simulink library "Linkage_Uprights"  (R2025a)
settings: Solver=VariableStepAuto  StartTime=0.0  StopTime=10.0  RelTol=1e-3
undefined symbols (not defined in the file): acamber, atoe, axle_len, axle_mass, axle_whlc_to_bearing, clr_axle, clr_conn_upr, clr_upr, hp_out_c_la, hp_out_f_la, hp_out_f_ua, hp_out_la, hp_out_r_la, hp_out_r_ua, hp_out_ua, hp_pushrod_out, hp_spr_bot, hp_upr_arb, hp_upr_cg, hp_upr_rod, hp_upr_wc, opc_axle, opc_conn_upr, opc_upr, radius_axle, radius_upr, size_conn_upr, upr_mass, whl_init_spd, X, Y, Z
libraries: sm_lib x147, Suspension_Utilities x50, fl_lib x9, nesl_utility x9
(part 1 of 5)
Description:
  | Component of Simscape Vehicle Templates Library
  | 
  | Copyright 2018-2026 The MathWorks, Inc.
settings Model: Creator=smiller  LastModifiedBy=smiller
settings SolverCC: AlgebraicLoopSolver=TrustRegion
settings DataIOCC: ReturnWorkspaceOutputs=off
settings OptimizationCC: ReuseModelBlockBuffer=off
settings DebuggingCC: UnconnectedInputMsg=warning  UnconnectedOutputMsg=warning  UnconnectedLineMsg=warning  ArithmeticOperatorsInVariantConditions=warning
settings ModelReferenceCC: EnableRefExpFcnMdlSchedulingChecks=on
settings SFSimCC: CustomCodeUndefinedFunction=UseInterfaceOnly
settings RTWCC: GPUComputeCapability=3.5

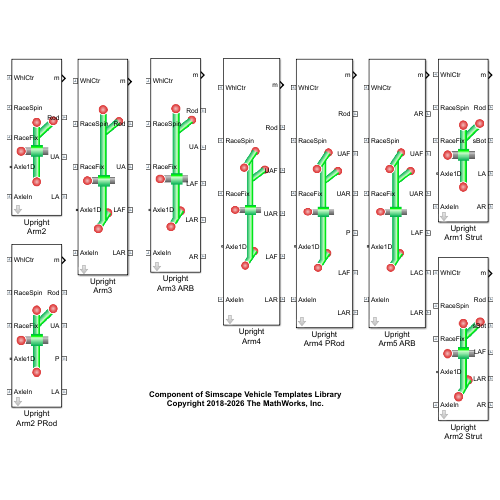
[thumbnail: Simulink's stored preview of the top-level diagram]
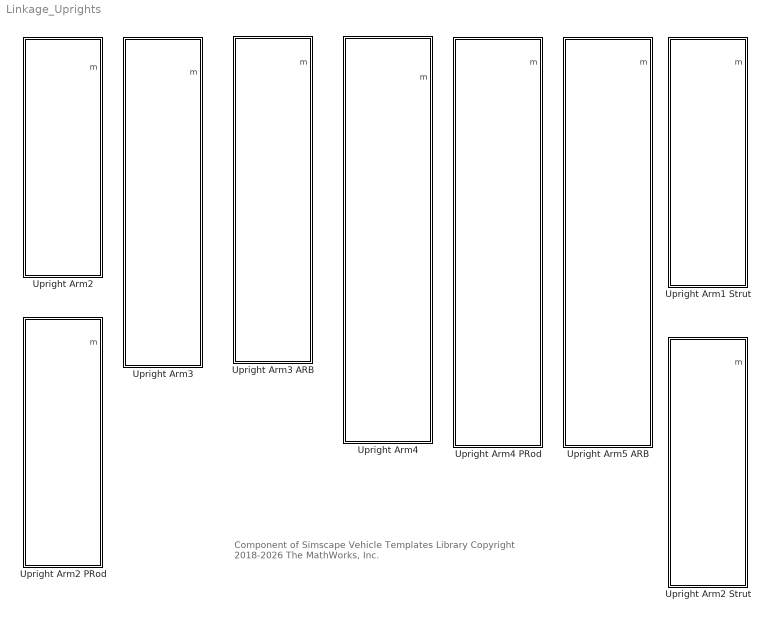
== system Linkage_Uprights ==
  note: Component of Simscape Vehicle Templates Library
      | Copyright 2018-2026 The MathWorks, Inc.
  Upright Arm1 Strut : Subsystem  mask(Upright for One Arm, Steering Rod, and Strut){popup_leftRight=Left, hp_spr_bot=hp_spr_bot, hp_la_out=hp_out_la, hp_upr_rod=hp_upr_rod, hp_upr_arb=hp_upr_arb, hp_upr_cg=hp_upr_cg, hp_upr_wc=hp_upr_wc, axle_len=axle_len, axle_whlc_to_bearing=axle_whlc_to_bearing, axle_mass=axle_mass, atoe=atoe, acamber=acamber, upr_mass=upr_mass, whl_init_spd_upr=whl_init_spd, clr_conn_upr=clr_conn_upr, opc_conn_upr=opc_conn_upr, size_conn_upr=size_conn_upr, clr_upr=clr_upr, opc_upr=opc_upr, radius_upr=radius_upr, clr_axle=clr_axle, opc_axle=opc_axle, radius_axle=radius_axle}
      mask prompts: popup_leftRight "Left/Right"; hp_spr_bot "Spring Bottom [xyz] (m)"; hp_la_out "Lower Arm Outboard [xyz] (m)"; hp_upr_rod "Track Rod Outboard [xyz] (m)"; hp_upr_arb "Anti-Roll Bar [xyz] (m)"; hp_upr_cg "Center of Mass [xyz] (m)"; hp_upr_wc "Wheel Center [xyz] (m)"; axle_len "Axle Length (m)"; axle_whlc_to_bearing "Distance Wheel Ctr to Bearing (m)"; axle_mass "Axle Mass (kg)"; atoe "Toe Angle (deg)"; acamber "Camber Angle (deg)"; upr_mass "Upright Mass (kg)"; whl_init_spd_upr "Initial Wheel Speed (rad/s)"
      mask help: Models an upright (or wheel carrier) that can connect to one arm, steering rod, and a strut. A strut (shock) will typically connect this to the chassis and constrain it to rotate about an axis.
      mask init:
      | % Set parameter for mirroring (+y or -y)
      | if(popup_leftRight == 1)
      |     rhs_upr = 1;
      | elseif(popup_leftRight == 2)
      |     rhs_upr = -1;
      | end
      | rhs_hp = [1 rhs_upr 1];
      | 
      | % Additional hardpoint at center of upright
      | % Used as attachment points for axle and steering arm
      | hp_upr_ctr = (hp_spr_bot+hp_la_out)/2;
      mask TypeOptions popup_leftRight: Left | Right
      mask TypeOptions axle_mass: Axle/Mass
      mask TypeOptions upr_mass:
      | Inertia
      | CG/Mass
      mask TypeOptions whl_init_spd_upr: Revolute/whl_init_spd_jnt
      mask TypeOptions clr_conn_upr:
      | Vis Upright LA/GraphicDiffuseColor | Vis Upright UA/GraphicDiffuseColor | Vis Wheel
      | Center/GraphicDiffuseColor
      mask TypeOptions opc_conn_upr:
      | Vis Upright LA/GraphicOpacity | Vis Upright UA/GraphicOpacity | Vis Wheel
      | Center/GraphicOpacity
      mask TypeOptions clr_upr:
      | Upright/clr_solid | Steering Arm/clr_solid | Bearing
      | Carrier/GraphicDiffuseColor
      mask TypeOptions opc_upr: Upright/opc_solid | Steering Arm/opc_solid
      mask TypeOptions radius_upr: Upright/rad_solid | Steering Arm/rad_solid
      mask TypeOptions clr_axle: Axle/GraphicDiffuseColor
      mask TypeOptions opc_axle: Axle/GraphicOpacity
      mask TypeOptions radius_axle: Axle/CylinderRadius
      mask DialogControl cont_upright Prompt: Upright
      mask DialogControl grp_init Prompt: Initialization
      mask DialogControl cont_vis_upr Prompt: Visualization
      mask DialogControl text_clr_upr Prompt: Color [RGB]
      mask DialogControl text_opc_upr Prompt: Opac. (0-1)
      mask DialogControl text_size_upr Prompt: Size (m)
      mask DialogControl text_conn_upr Prompt: Connections
      mask DialogControl text_upright Prompt: Upright
      mask DialogControl text_stub_axle Prompt: Axle
      mask Display: image('sm_car_vehicle_linkage_dw_upr_IMAGE.png');
  Upright Arm2 : Subsystem  mask(Upright for Two Arms and Steering Rod){popup_leftRight=Left, hp_ua_out=hp_out_ua, hp_la_out=hp_out_la, hp_upr_rod=hp_upr_rod, hp_upr_cg=hp_upr_cg, hp_upr_wc=hp_upr_wc, axle_len=axle_len, axle_whlc_to_bearing=axle_whlc_to_bearing, axle_mass=axle_mass, atoe=atoe, acamber=acamber, upr_mass=upr_mass, whl_init_spd_upr=whl_init_spd, clr_conn_upr=clr_conn_upr, opc_conn_upr=opc_conn_upr, size_conn_upr=size_conn_upr, clr_upr=clr_upr, opc_upr=opc_upr, radius_upr=radius_upr, clr_axle=clr_axle, opc_axle=opc_axle, radius_axle=radius_axle}
      mask prompts: popup_leftRight "Left/Right"; hp_ua_out "Upper Arm Outboard [xyz] (m)"; hp_la_out "Lower Arm Outboard [xyz] (m)"; hp_upr_rod "Track Rod Outboard [xyz] (m)"; hp_upr_cg "Center of Mass [xyz] (m)"; hp_upr_wc "Wheel Center [xyz] (m)"; axle_len "Axle Length (m)"; axle_whlc_to_bearing "Distance Wheel Ctr to Bearing (m)"; axle_mass "Axle Mass (kg)"; atoe "Toe Angle (deg)"; acamber "Camber Angle (deg)"; upr_mass "Upright Mass (kg)"; whl_init_spd_upr "Initial Wheel Speed (rad/s)"
      mask help: Models an upright (or wheel carrier) that can connect to two arms and a steering rod.
      mask init:
      | % Set parameter for mirroring (+y or -y)
      | if(popup_leftRight == 1)
      |     rhs_upr = 1;
      | elseif(popup_leftRight == 2)
      |     rhs_upr = -1;
      | end
      | rhs_hp = [1 rhs_upr 1];
      | 
      | % Additional hardpoint at center of upright
      | % Used as attachment points for axle and steering arm
      | hp_upr_ctr = (hp_ua_out+hp_la_out)/2;
      mask TypeOptions popup_leftRight: Left | Right
      mask TypeOptions axle_mass: Axle/Mass
      mask TypeOptions upr_mass:
      | Inertia
      | CG/Mass
      mask TypeOptions whl_init_spd_upr: Revolute/whl_init_spd_jnt
      mask TypeOptions clr_conn_upr:
      | Vis Upright LA/GraphicDiffuseColor | Vis Upright UA/GraphicDiffuseColor | Vis Wheel
      | Center/GraphicDiffuseColor
      mask TypeOptions opc_conn_upr:
      | Vis Upright LA/GraphicOpacity | Vis Upright UA/GraphicOpacity | Vis Wheel
      | Center/GraphicOpacity
      mask TypeOptions clr_upr: Upright/clr_solid | Steering Arm/clr_solid
      mask TypeOptions opc_upr: Upright/opc_solid | Steering Arm/opc_solid
      mask TypeOptions radius_upr: Upright/rad_solid | Steering Arm/rad_solid
      mask TypeOptions clr_axle: Axle/GraphicDiffuseColor
      mask TypeOptions opc_axle: Axle/GraphicOpacity
      mask TypeOptions radius_axle: Axle/CylinderRadius
      mask DialogControl cont_upright Prompt: Upright
      mask DialogControl grp_upright Prompt: Initialization
      mask DialogControl cont_vis_upr Prompt: Visualization
      mask DialogControl text_clr_upr Prompt: Color [RGB]
      mask DialogControl text_opc_upr Prompt: Opac. (0-1)
      mask DialogControl text_size_upr Prompt: Size (m)
      mask DialogControl text_conn_upr Prompt: Connections
      mask DialogControl text_upright Prompt: Upright
      mask DialogControl text_axle Prompt: Axle
      mask Display: image('sm_car_vehicle_linkage_dw_upr_IMAGE.png');
  Upright Arm2 PRod : Subsystem  mask(Upright for Two Arms, Steering Rod, and Pushrod){popup_leftRight=Left, hp_ua_out=hp_out_ua, hp_la_out=hp_out_la, hp_upr_rod=hp_upr_rod, hp_pushrod=hp_pushrod_out, hp_upr_cg=hp_upr_cg, hp_upr_wc=hp_upr_wc, axle_len=axle_len, axle_whlc_to_bearing=axle_whlc_to_bearing, axle_mass=axle_mass, atoe=atoe, acamber=acamber, upr_mass=upr_mass, whl_init_spd_upr=whl_init_spd, clr_conn_upr=clr_conn_upr, opc_conn_upr=opc_conn_upr, size_conn_upr=size_conn_upr, clr_upr=clr_upr, opc_upr=opc_upr, radius_upr=radius_upr, clr_axle=clr_axle, opc_axle=opc_axle, radius_axle=radius_axle}
      mask prompts: popup_leftRight "Left/Right"; hp_ua_out "Upper Arm Outboard [xyz] (m)"; hp_la_out "Lower Arm Outboard [xyz] (m)"; hp_upr_rod "Track Rod Outboard [xyz] (m)"; hp_pushrod "Pushrod Outboard [xyz] (m)"; hp_upr_cg "Center of Mass [xyz] (m)"; hp_upr_wc "Wheel Center [xyz] (m)"; axle_len "Axle Length (m)"; axle_whlc_to_bearing "Distance Wheel Ctr to Bearing (m)"; axle_mass "Axle Mass (kg)"; atoe "Toe Angle (deg)"; acamber "Camber Angle (deg)"; upr_mass "Upright Mass (kg)"; whl_init_spd_upr "Initial Wheel Speed (rad/s)"
      mask help: Models an upright (or wheel carrier) that can connect to two arms, a steering rod, and a pushrod.
      mask init:
      | % Set parameter for mirroring (+y or -y)
      | if(popup_leftRight == 1)
      |     rhs_upr = 1;
      | elseif(popup_leftRight == 2)
      |     rhs_upr = -1;
      | end
      | rhs_hp = [1 rhs_upr 1];
      | 
      | % Additional hardpoint at center of upright
      | % Used as attachment points for axle and steering arm
      | hp_upr_ctr = (hp_ua_out+hp_la_out)/2;
      mask TypeOptions popup_leftRight: Left | Right
      mask TypeOptions axle_mass: Axle/Mass
      mask TypeOptions upr_mass:
      | Inertia
      | CG/Mass
      mask TypeOptions whl_init_spd_upr: Revolute/whl_init_spd_jnt
      mask TypeOptions clr_conn_upr:
      | Vis Upright LA/GraphicDiffuseColor | Vis Upright UA/GraphicDiffuseColor | Vis Wheel
      | Center/GraphicDiffuseColor
      mask TypeOptions opc_conn_upr:
      | Vis Upright LA/GraphicOpacity | Vis Upright UA/GraphicOpacity | Vis Wheel
      | Center/GraphicOpacity
      mask TypeOptions clr_upr:
      | Upright/clr_solid | Steering Arm/clr_solid | Bearing
      | Carrier/GraphicDiffuseColor | Pushrod Conn/clr_solid
      mask TypeOptions opc_upr: Upright/opc_solid | Steering Arm/opc_solid | Pushrod Conn/opc_solid
      mask TypeOptions radius_upr: Upright/rad_solid | Steering Arm/rad_solid | Pushrod Conn/rad_solid
      mask TypeOptions clr_axle: Axle/GraphicDiffuseColor
      mask TypeOptions opc_axle: Axle/GraphicOpacity
      mask TypeOptions radius_axle: Axle/CylinderRadius
      mask DialogControl cont_upright Prompt: Upright
      mask DialogControl grp_init Prompt: Initialization
      mask DialogControl cont_vis_upr Prompt: Visualization
      mask DialogControl text_clr_upr Prompt: Color [RGB]
      mask DialogControl text_opc_upr Prompt: Opac. (0-1)
      mask DialogControl text_size_upr Prompt: Size (m)
      mask DialogControl text_conn_upr Prompt: Connections
      mask DialogControl text_upright Prompt: Upright
      mask DialogControl text_stub_axle Prompt: Axle
      mask Display: image('sm_car_vehicle_linkage_dw_upr_IMAGE.png');
  Upright Arm2 Strut : Subsystem  mask(Upright for Two Arms, Steering Rod, and Strut){popup_leftRight=Left, hp_spr_bot=hp_spr_bot, hp_laf_out=hp_out_f_la, hp_lar_out=hp_out_r_la, hp_upr_rod=hp_upr_rod, hp_upr_arb=hp_upr_arb, hp_upr_cg=hp_upr_cg, hp_upr_wc=hp_upr_wc, axle_len=axle_len, axle_whlc_to_bearing=axle_whlc_to_bearing, axle_mass=axle_mass, atoe=atoe, acamber=acamber, upr_mass=upr_mass, whl_init_spd_upr=whl_init_spd, clr_conn_upr=clr_conn_upr, opc_conn_upr=opc_conn_upr, size_conn_upr=size_conn_upr, clr_upr=clr_upr, opc_upr=opc_upr, radius_upr=radius_upr, clr_axle=clr_axle, opc_axle=opc_axle, radius_axle=radius_axle}
      mask prompts: popup_leftRight "Left/Right"; hp_spr_bot "Spring Bottom [xyz] (m)"; hp_laf_out "Lower Arm Front Outboard [xyz] (m)"; hp_lar_out "Lower Arm Rear Outboard [xyz] (m)"; hp_upr_rod "Track Rod Outboard [xyz] (m)"; hp_upr_arb "Anti-Roll Bar [xyz] (m)"; hp_upr_cg "Center of Mass [xyz] (m)"; hp_upr_wc "Wheel Center [xyz] (m)"; axle_len "Axle Length (m)"; axle_whlc_to_bearing "Distance Wheel Ctr to Bearing (m)"; axle_mass "Axle Mass (kg)"; atoe "Toe Angle (deg)"; acamber "Camber Angle (deg)"; upr_mass "Upright Mass (kg)"; whl_init_spd_upr "Initial Wheel Speed (rad/s)"
      mask help: Models an upright (or wheel carrier) that can connect to two arms, steering rod, and a strut. A strut (shock) will typically connect this to the chassis and constrain it to rotate about an axis.
      mask init:
      | % Set parameter for mirroring (+y or -y)
      | if(popup_leftRight == 1)
      |     rhs_upr = 1;
      | elseif(popup_leftRight == 2)
      |     rhs_upr = -1;
      | end
      | rhs_hp = [1 rhs_upr 1];
      | 
      | % Additional hardpoint at center of upright
      | % Used as attachment points for axle and steering arm
      | hp_upr_ctr = (hp_spr_bot+hp_laf_out)/2;
      mask TypeOptions popup_leftRight: Left | Right
      mask TypeOptions axle_mass: Axle/Mass
      mask TypeOptions upr_mass:
      | Inertia
      | CG/Mass
      mask TypeOptions whl_init_spd_upr: Revolute/whl_init_spd_jnt
      mask TypeOptions clr_conn_upr:
      | Vis Upright LA/GraphicDiffuseColor | Vis Upright UA/GraphicDiffuseColor | Vis Wheel
      | Center/GraphicDiffuseColor
      mask TypeOptions opc_conn_upr:
      | Vis Upright LA/GraphicOpacity | Vis Upright UA/GraphicOpacity | Vis Wheel
      | Center/GraphicOpacity
      mask TypeOptions clr_upr:
      | Upright/clr_solid | Steering Arm/clr_solid | Bearing
      | Carrier/GraphicDiffuseColor
      mask TypeOptions opc_upr: Upright/opc_solid | Steering Arm/opc_solid
      mask TypeOptions radius_upr: Upright/rad_solid | Steering Arm/rad_solid
      mask TypeOptions clr_axle: Axle/GraphicDiffuseColor
      mask TypeOptions opc_axle: Axle/GraphicOpacity
      mask TypeOptions radius_axle: Axle/CylinderRadius
      mask DialogControl cont_upright Prompt: Upright
      mask DialogControl grp_init Prompt: Initialization
      mask DialogControl cont_vis_upr Prompt: Visualization
      mask DialogControl text_clr_upr Prompt: Color [RGB]
      mask DialogControl text_opc_upr Prompt: Opac. (0-1)
      mask DialogControl text_size_upr Prompt: Size (m)
      mask DialogControl text_conn_upr Prompt: Connections
      mask DialogControl text_upright Prompt: Upright
      mask DialogControl text_stub_axle Prompt: Axle
      mask Display: image('sm_car_vehicle_linkage_sla_arb_IMAGE.png');
  Upright Arm3 : Subsystem  mask(Upright for Three Arms and Steering Rod){popup_leftRight=Left, hp_ua_out=hp_out_ua, hp_laf_out=hp_out_f_la, hp_lar_out=hp_out_r_la, hp_upr_rod=hp_upr_rod, hp_upr_cg=hp_upr_cg, hp_upr_wc=hp_upr_wc, axle_len=axle_len, axle_whlc_to_bearing=axle_whlc_to_bearing, axle_mass=axle_mass, atoe=atoe, acamber=acamber, upr_mass=upr_mass, whl_init_spd_upr=whl_init_spd, clr_conn_upr=clr_conn_upr, opc_conn_upr=opc_conn_upr, size_conn_upr=size_conn_upr, clr_upr=clr_upr, opc_upr=opc_upr, radius_upr=radius_upr, clr_axle=clr_axle, opc_axle=opc_axle, radius_axle=radius_axle}
      mask prompts: popup_leftRight "Left/Right"; hp_ua_out "Upper Arm Outboard [xyz] (m)"; hp_laf_out "Lower Front Arm Outboard [xyz] (m)"; hp_lar_out "Lower Rear Arm Outboard [xyz] (m)"; hp_upr_rod "Track Rod Outboard [xyz] (m)"; hp_upr_cg "Center of Mass [xyz] (m)"; hp_upr_wc "Wheel Center [xyz] (m)"; axle_len "Axle Length(m)"; axle_whlc_to_bearing "Distance Wheel Ctr to Bearing (m)"; axle_mass "Axle Mass (kg)"; atoe "Toe Angle (deg)"; acamber "Camber Angle (deg)"; upr_mass "Upright Mass (kg)"; whl_init_spd_upr "Initial Wheel Speed (rad/s)"
      mask help: Models an upright (or wheel carrier) that can connect to three arms and a steering rod.
      mask init:
      | % Set parameter for mirroring (+y or -y)
      | if(popup_leftRight == 1)
      |     rhs_upr = 1;
      | elseif(popup_leftRight == 2)
      |     rhs_upr = -1;
      | end
      | rhs_hp = [1 rhs_upr 1];
      | 
      | % Additional hardpoint at center of upright
      | % Used as attachment points for axle and steering arm
      | hp_upr_ctr = (hp_ua_out+hp_laf_out)/2;
      mask TypeOptions popup_leftRight: Left | Right
      mask TypeOptions axle_mass: Axle/Mass
      mask TypeOptions upr_mass:
      | Inertia
      | CG/Mass
      mask TypeOptions whl_init_spd_upr: Revolute/whl_init_spd_jnt
      mask TypeOptions clr_conn_upr:
      | Vis Upright LAF/GraphicDiffuseColor | Vis Upright UAF/GraphicDiffuseColor | Vis Wheel
      | Center/GraphicDiffuseColor
      mask TypeOptions opc_conn_upr:
      | Vis Upright LAF/GraphicOpacity | Vis Upright UAF/GraphicOpacity | Vis Wheel
      | Center/GraphicOpacity
      mask TypeOptions clr_upr: Upright/clr_solid | Steering Arm/clr_solid
      mask TypeOptions opc_upr: Upright/opc_solid | Steering Arm/opc_solid
      mask TypeOptions radius_upr: Upright/rad_solid | Steering Arm/rad_solid
      mask TypeOptions clr_axle: Axle/GraphicDiffuseColor
      mask TypeOptions opc_axle: Axle/GraphicOpacity
      mask TypeOptions radius_axle: Axle/CylinderRadius
      mask DialogControl cont_upright Prompt: Upright
      mask DialogControl grp_upright Prompt: Upright
      mask DialogControl cont_vis_upr Prompt: Visualization
      mask DialogControl text_clr_upr Prompt: Color [RGB]
      mask DialogControl text_opc_upr Prompt: Opac. (0-1)
      mask DialogControl text_size_upr Prompt: Size (m)
      mask DialogControl text_conn_upr Prompt: Connections
      mask DialogControl text_upright Prompt: Upright
      mask DialogControl text_axle Prompt: Axle
      mask Display: image('sm_car_vehicle_linkage_sla_upr_IMAGE.png');
  Upright Arm3 ARB : Subsystem  mask(Upright for Three Arms, Steering Rod, Anti-Roll Bar){popup_leftRight=Left, hp_ua_out=hp_out_ua, hp_laf_out=hp_out_f_la, hp_lar_out=hp_out_r_la, hp_upr_rod=hp_upr_rod, hp_upr_arb=hp_upr_arb, hp_upr_cg=hp_upr_cg, hp_upr_wc=hp_upr_wc, axle_len=axle_len, axle_whlc_to_bearing=axle_whlc_to_bearing, axle_mass=axle_mass, atoe=atoe, acamber=acamber, upr_mass=upr_mass, whl_init_spd_upr=whl_init_spd, clr_conn_upr=clr_conn_upr, opc_conn_upr=opc_conn_upr, size_conn_upr=size_conn_upr, clr_upr=clr_upr, opc_upr=opc_upr, radius_upr=radius_upr, clr_axle=clr_axle, opc_axle=opc_axle, radius_axle=radius_axle}
      mask prompts: popup_leftRight "Left/Right"; hp_ua_out "Upper Arm Outboard [xyz] (m)"; hp_laf_out "Lower Front Arm Outboard [xyz] (m)"; hp_lar_out "Lower Rear Arm Outboard [xyz] (m)"; hp_upr_rod "Track Rod Outboard [xyz] (m)"; hp_upr_arb "Anti-Roll Bar [xyz] (m)"; hp_upr_cg "Center of Mass [xyz] (m)"; hp_upr_wc "Wheel Center [xyz] (m)"; axle_len "Axle Length(m)"; axle_whlc_to_bearing "Distance Wheel Ctr to Bearing (m)"; axle_mass "Axle Mass (kg)"; atoe "Toe Angle (deg)"; acamber "Camber Angle (deg)"; upr_mass "Upright Mass (kg)"; whl_init_spd_upr "Initial Wheel Speed (rad/s)"
      mask help: Models an upright (or wheel carrier) that can connect to three arms, a steering rod and an anti-roll bar.
      mask init: same as Linkage_Uprights/Upright Arm3
      mask TypeOptions popup_leftRight: Left | Right
      mask TypeOptions axle_mass: Axle/Mass
      mask TypeOptions upr_mass:
      | Inertia
      | CG/Mass
      mask TypeOptions whl_init_spd_upr: Revolute/whl_init_spd_jnt
      mask TypeOptions clr_conn_upr:
      | Vis Upright LAF/GraphicDiffuseColor | Vis Upright UAF/GraphicDiffuseColor | Vis Wheel
      | Center/GraphicDiffuseColor
      mask TypeOptions opc_conn_upr:
      | Vis Upright LAF/GraphicOpacity | Vis Upright UAF/GraphicOpacity | Vis Wheel
      | Center/GraphicOpacity
      mask TypeOptions clr_upr: Upright/clr_solid | Steering Arm/clr_solid
      mask TypeOptions opc_upr: Upright/opc_solid | Steering Arm/opc_solid
      mask TypeOptions radius_upr: Upright/rad_solid | Steering Arm/rad_solid
      mask TypeOptions clr_axle: Axle/GraphicDiffuseColor
      mask TypeOptions opc_axle: Axle/GraphicOpacity
      mask TypeOptions radius_axle: Axle/CylinderRadius
      mask DialogControl cont_upright Prompt: Upright
      mask DialogControl grp_upright Prompt: Upright
      mask DialogControl cont_vis_upr Prompt: Visualization
      mask DialogControl text_clr_upr Prompt: Color [RGB]
      mask DialogControl text_opc_upr Prompt: Opac. (0-1)
      mask DialogControl text_size_upr Prompt: Size (m)
      mask DialogControl text_conn_upr Prompt: Connections
      mask DialogControl text_upright Prompt: Upright
      mask DialogControl text_axle Prompt: Axle
      mask Display: image('sm_car_vehicle_linkage_sla_upr_IMAGE.png');
  Upright Arm4 : Subsystem  mask(Upright for Four Arms and Steering Rod){popup_leftRight=Left, hp_uaf_out=hp_out_f_ua, hp_uar_out=hp_out_r_ua, hp_laf_out=hp_out_f_la, hp_lar_out=hp_out_r_la, hp_upr_rod=hp_upr_rod, hp_upr_cg=hp_upr_cg, hp_upr_wc=hp_upr_wc, axle_len=axle_len, axle_whlc_to_bearing=axle_whlc_to_bearing, axle_mass=axle_mass, atoe=atoe, acamber=acamber, upr_mass=upr_mass, whl_init_spd_upr=whl_init_spd, clr_conn_upr=clr_conn_upr, opc_conn_upr=opc_conn_upr, size_conn_upr=size_conn_upr, clr_upr=clr_upr, opc_upr=opc_upr, radius_upr=radius_upr, clr_axle=clr_axle, opc_axle=opc_axle, radius_axle=radius_axle}
      mask prompts: popup_leftRight "Left/Right"; hp_uaf_out "Upper Arm Front Outboard [xyz] (m)"; hp_uar_out "Upper Arm Rear Outboard [xyz] (m)"; hp_laf_out "Lower Arm Front Outboard [xyz] (m)"; hp_lar_out "Lower Arm Rear Outboard [xyz] (m)"; hp_upr_rod "Track Rod Outboard [xyz] (m)"; hp_upr_cg "Center of Mass [xyz] (m)"; hp_upr_wc "Wheel Center [xyz] (m)"; axle_len "Axle Length (m)"; axle_whlc_to_bearing "Distance Wheel Ctr to Bearing (m)"; axle_mass "Axle Mass (kg)"; atoe "Toe Angle (deg)"; acamber "Camber Angle (deg)"; upr_mass "Upright Mass (kg)"; whl_init_spd_upr "Initial Wheel Speed (rad/s)"
      mask help: Models an upright (or wheel carrier) that can connect to four arms and a steering rod.
      mask init:
      | % Set parameter for mirroring (+y or -y)
      | if(popup_leftRight == 1)
      |     rhs_upr = 1;
      | elseif(popup_leftRight == 2)
      |     rhs_upr = -1;
      | end
      | rhs_hp = [1 rhs_upr 1];
      | 
      | % Additional hardpoint at center of upright
      | % Used as attachment points for axle and steering arm
      | hp_upr_ctr = (hp_uaf_out+hp_laf_out)/2;
      mask TypeOptions popup_leftRight: Left | Right
      mask TypeOptions axle_mass: Axle/Mass
      mask TypeOptions upr_mass:
      | Inertia
      | CG/Mass
      mask TypeOptions whl_init_spd_upr: Revolute/whl_init_spd_jnt
      mask TypeOptions clr_conn_upr:
      | Vis Upright LAF/GraphicDiffuseColor | Vis Upright UAF/GraphicDiffuseColor | Vis
      | Wheel
      | Center/GraphicDiffuseColor
      mask TypeOptions opc_conn_upr:
      | Vis Upright LAF/GraphicOpacity | Vis Upright UAF/GraphicOpacity | Vis
      | Wheel
      | Center/GraphicOpacity
      mask TypeOptions clr_upr: Upright/clr_solid | Steering Arm/clr_solid
      mask TypeOptions opc_upr: Upright/opc_solid | Steering Arm/opc_solid
      mask TypeOptions radius_upr: Upright/rad_solid | Steering Arm/rad_solid
      mask TypeOptions clr_axle: Axle/GraphicDiffuseColor
      mask TypeOptions opc_axle: Axle/GraphicOpacity
      mask TypeOptions radius_axle: Axle/CylinderRadius
      mask DialogControl cont_upright Prompt: Upright
      mask DialogControl grp_upright Prompt: Initialization
      mask DialogControl cont_vis_upr Prompt: Visualization
      mask DialogControl text_clr_upr Prompt: Color [RGB]
      mask DialogControl text_opc_upr Prompt: Opac. (0-1)
      mask DialogControl text_size_upr Prompt: Size (m)
      mask DialogControl text_conn_upr Prompt: Connections
      mask DialogControl text_upright Prompt: Upright
      mask DialogControl text_axle Prompt: Axle
      mask Display: image('sm_car_vehicle_linkage_link5_upr_IMAGE.png');
  Upright Arm4 PRod : Subsystem  mask(Upright for Four Arms, Steering Rod, and Pushrod){popup_leftRight=Left, hp_uaf_out=hp_out_f_ua, hp_uar_out=hp_out_r_ua, hp_laf_out=hp_out_f_la, hp_lar_out=hp_out_r_la, hp_pushrod=hp_pushrod_out, hp_upr_rod=hp_upr_rod, hp_upr_cg=hp_upr_cg, hp_upr_wc=hp_upr_wc, axle_len=axle_len, axle_whlc_to_bearing=axle_whlc_to_bearing, axle_mass=axle_mass, atoe=atoe, acamber=acamber, upr_mass=upr_mass, whl_init_spd_upr=whl_init_spd, clr_conn_upr=clr_conn_upr, opc_conn_upr=opc_conn_upr, size_conn_upr=size_conn_upr, clr_upr=clr_upr, opc_upr=opc_upr, radius_upr=radius_upr, clr_axle=clr_axle, opc_axle=opc_axle, radius_axle=radius_axle}
      mask prompts: popup_leftRight "Left/Right"; hp_uaf_out "Upper Arm Front Outboard [xyz] (m)"; hp_uar_out "Upper Arm Rear Outboard [xyz] (m)"; hp_laf_out "Lower Arm Front Outboard [xyz] (m)"; hp_lar_out "Lower Arm Rear Outboard [xyz] (m)"; hp_pushrod "Pushrod Outboard [xyz] (m)"; hp_upr_rod "Track Rod Outboard [xyz] (m)"; hp_upr_cg "Center of Mass [xyz] (m)"; hp_upr_wc "Wheel Center [xyz] (m)"; axle_len "Axle Length (m)"; axle_whlc_to_bearing "Distance Wheel Ctr to Bearing (m)"; axle_mass "Axle Mass (kg)"; atoe "Toe Angle (deg)"; acamber "Camber Angle (deg)"; upr_mass "Upright Mass (kg)"; whl_init_spd_upr "Initial Wheel Speed (rad/s)"
      mask help: Models an upright (or wheel carrier) that can connect to four arms, a steering rod, and a pushrod.
      mask init: same as Linkage_Uprights/Upright Arm4
      mask TypeOptions popup_leftRight: Left | Right
      mask TypeOptions axle_mass: Axle/Mass
      mask TypeOptions upr_mass:
      | Inertia
      | CG/Mass
      mask TypeOptions whl_init_spd_upr: Revolute/whl_init_spd_jnt
      mask TypeOptions clr_conn_upr:
      | Vis Upright LAF/GraphicDiffuseColor | Vis Upright UAF/GraphicDiffuseColor | Vis
      | Wheel
      | Center/GraphicDiffuseColor
      mask TypeOptions opc_conn_upr:
      | Vis Upright LAF/GraphicOpacity | Vis Upright UAF/GraphicOpacity | Vis
      | Wheel
      | Center/GraphicOpacity
      mask TypeOptions clr_upr:
      | Upright/clr_solid | Steering Arm/clr_solid | Lower
      | Rear Arm/clr_solid | Upper
      | Rear Arm/clr_solid | Pushrod Conn/clr_solid
      mask TypeOptions opc_upr:
      | Upright/opc_solid | Steering Arm/opc_solid | Lower
      | Rear Arm/opc_solid | Upper
      | Rear Arm/opc_solid | Pushrod Conn/opc_solid
      mask TypeOptions radius_upr:
      | Upright/rad_solid | Steering Arm/rad_solid | Lower
      | Rear Arm/rad_solid | Upper
      | Rear Arm/rad_solid | Pushrod Conn/rad_solid
      mask TypeOptions clr_axle: Axle/GraphicDiffuseColor
      mask TypeOptions opc_axle: Axle/GraphicOpacity
      mask TypeOptions radius_axle: Axle/CylinderRadius
      mask DialogControl cont_upright Prompt: Upright
      mask DialogControl grp_upright Prompt: Initialization
      mask DialogControl cont_vis_upr Prompt: Visualization
      mask DialogControl text_clr_upr Prompt: Color [RGB]
      mask DialogControl text_opc_upr Prompt: Opac. (0-1)
      mask DialogControl text_size_upr Prompt: Size (m)
      mask DialogControl text_conn_upr Prompt: Connections
      mask DialogControl text_upright Prompt: Upright
      mask DialogControl text_axle Prompt: Axle
      mask Display: image('sm_car_vehicle_linkage_link5_upr_IMAGE.png');
  Upright Arm5 ARB : Subsystem  mask(Upright for Five Arms and an Anti-Roll Bar){popup_leftRight=Left, hp_uaf_out=hp_out_f_ua, hp_uar_out=hp_out_r_ua, hp_laf_out=hp_out_f_la, hp_lar_out=hp_out_r_la, hp_lac_out=hp_out_c_la, hp_arb=hp_upr_arb, hp_upr_cg=hp_upr_cg, hp_upr_wc=hp_upr_wc, axle_len=axle_len, axle_whlc_to_bearing=axle_whlc_to_bearing, axle_mass=axle_mass, atoe=atoe, acamber=acamber, upr_mass=upr_mass, whl_init_spd_upr=whl_init_spd, clr_conn_upr=clr_conn_upr, opc_conn_upr=opc_conn_upr, size_conn_upr=size_conn_upr, clr_upr=clr_upr, opc_upr=opc_upr, radius_upr=radius_upr, clr_axle=clr_axle, opc_axle=opc_axle, radius_axle=radius_axle}
      mask prompts: popup_leftRight "Left/Right"; hp_uaf_out "Upper Arm Front Outboard [xyz] (m)"; hp_uar_out "Upper Arm Rear Outboard [xyz] (m)"; hp_laf_out "Lower Arm Front Outboard [xyz] (m)"; hp_lar_out "Lower Arm Rear Outboard [xyz] (m)"; hp_lac_out "Lower Arm Center Outboard [xyz] (m)"; hp_arb "Anti-Roll Bar [xyz] (m)"; hp_upr_cg "Center of Mass [xyz] (m)"; hp_upr_wc "Wheel Center [xyz] (m)"; axle_len "Axle Length (m)"; axle_whlc_to_bearing "Distance Wheel Ctr to Bearing (m)"; axle_mass "Axle Mass (kg)"; atoe "Toe Angle (deg)"; acamber "Camber Angle (deg)"; upr_mass "Upright Mass (kg)"; whl_init_spd_upr "Initial Wheel Speed (rad/s)"
      mask help: Models an upright (or wheel carrier) that can connect to five arms and an anti-roll bar.
      mask init: same as Linkage_Uprights/Upright Arm4
      mask TypeOptions popup_leftRight: Left | Right
      mask TypeOptions axle_mass: Axle/Mass
      mask TypeOptions upr_mass:
      | Inertia
      | CG/Mass
      mask TypeOptions whl_init_spd_upr: Revolute/whl_init_spd_jnt
      mask TypeOptions clr_conn_upr:
      | Vis Upright LAF/GraphicDiffuseColor | Vis Upright UAF/GraphicDiffuseColor | Vis
      | Wheel
      | Center/GraphicDiffuseColor
      mask TypeOptions opc_conn_upr:
      | Vis Upright LAF/GraphicOpacity | Vis Upright UAF/GraphicOpacity | Vis
      | Wheel
      | Center/GraphicOpacity
      mask TypeOptions clr_upr:
      | Upright/clr_solid | ARB/clr_solid | Lower
      | Rear Arm/clr_solid | Upper
      | Rear Arm/clr_solid | Lower
      | Center Arm/clr_solid
      mask TypeOptions opc_upr:
      | Upright/opc_solid | ARB/opc_solid | Lower
      | Rear Arm/opc_solid | Upper
      | Rear Arm/opc_solid | Lower
      | Center Arm/opc_solid
      mask TypeOptions radius_upr:
      | Upright/rad_solid | ARB/rad_solid | Lower
      | Rear Arm/rad_solid | Upper
      | Rear Arm/rad_solid | Lower
      | Center Arm/rad_solid
      mask TypeOptions clr_axle: Axle/GraphicDiffuseColor
      mask TypeOptions opc_axle: Axle/GraphicOpacity
      mask TypeOptions radius_axle: Axle/CylinderRadius
      mask DialogControl cont_upright Prompt: Upright
      mask DialogControl grp_upright Prompt: Initialization
      mask DialogControl cont_vis_upr Prompt: Visualization
      mask DialogControl text_clr_upr Prompt: Color [RGB]
      mask DialogControl text_opc_upr Prompt: Opac. (0-1)
      mask DialogControl text_size_upr Prompt: Size (m)
      mask DialogControl text_conn_upr Prompt: Connections
      mask DialogControl text_upright Prompt: Upright
      mask DialogControl text_axle Prompt: Axle
      mask Display: image('sm_car_vehicle_linkage_link5_upr_IMAGE.png');

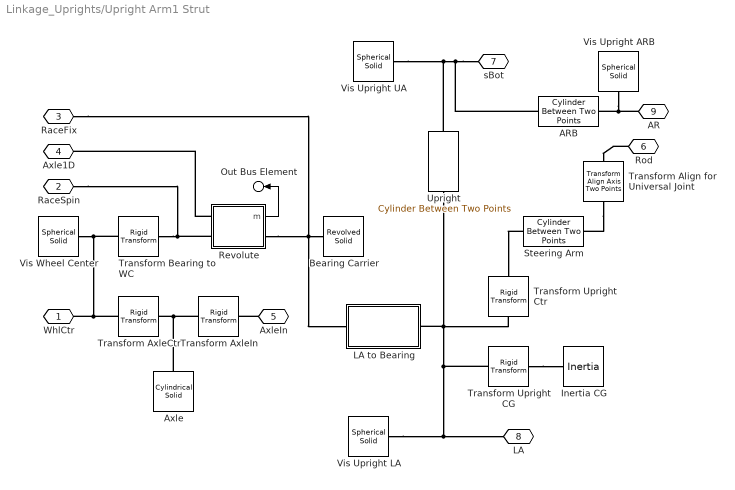
== system Linkage_Uprights/Upright Arm1 Strut ==
  ARB : Suspension_Utilities/Cylinder Between Two Points  hp_b=hp_spr_bot.*rhs_hp  hp_f=hp_upr_arb.*rhs_hp  Mass=0  clr_solid=clr_upr  opc_solid=opc_upr  rad_solid=radius_upr
  Axle : sm_lib/Body Elements/Cylindrical Solid  CylinderRadius=radius_axle  CylinderRadiusUnits=m  CylinderLength=axle_len  CylinderLengthUnits=m  ExportEntireGeometry=off  InertiaType=CalculateFromGeometry  BasedOnType=Mass  Density=7000  DensityUnits=kg/m^3  Mass=axle_mass  MassUnits=kg  CenterOfMass=[0 0 0]  CenterOfMassUnits=m  MomentsOfInertia=[1 1 1]  MomentsOfInertiaUnits=kg*m^2  ProductsOfInertia=[0 0 0]  ProductsOfInertiaUnits=kg*m^2  GraphicType=FromGeometry  MarkerShape=Sphere  MarkerSize=10  GraphicVisPropType=SimpleVisualProperties  GraphicDiffuseColor=clr_axle  GraphicOpacity=opc_axle  GraphicSpecularColor=[0.5 0.5 0.5 1.0]  GraphicAmbientColor=[0.15 0.15 0.15 1.0]  GraphicEmissiveColor=[0.0 0.0 0.0 1.0]  GraphicShininess=75  DoExposeReferenceFrame=on  SerializedFrames=<Frames/>
  Bearing Carrier : sm_lib/Body Elements/Revolved Solid  RevolutionCrossSection=[1.2 0.5;1.1 0.5;1.1 -0.5;1.2 -0.5].*[radius_axle 0.05]  RevolutionCrossSectionUnits=m  RevolutionExtent=Full  RevolutionAngle=180  RevolutionAngleUnits=deg  ExportConvexHullGeometry=off  InertiaType=CalculateFromGeometry  BasedOnType=Density  Density=1000  DensityUnits=kg/m^3  Mass=1  MassUnits=kg  CenterOfMass=[0 0 0]  CenterOfMassUnits=m  MomentsOfInertia=[1 1 1]  MomentsOfInertiaUnits=kg*m^2  ProductsOfInertia=[0 0 0]  ProductsOfInertiaUnits=kg*m^2  GraphicType=FromGeometry  MarkerShape=Sphere  MarkerSize=10  GraphicVisPropType=SimpleVisualProperties  GraphicDiffuseColor=clr_upr  GraphicOpacity=0.5  GraphicSpecularColor=[0.5 0.5 0.5 1.0]  GraphicAmbientColor=[0.15 0.15 0.15 1.0]  GraphicEmissiveColor=[0.0 0.0 0.0 1.0]  GraphicShininess=75  DoExposeReferenceFrame=on  SerializedFrames=<Frames/>
  Inertia CG : sm_lib/Body Elements/Inertia  InertiaType=PointMass  Mass=upr_mass  MassUnits=kg  CenterOfMass=[0 0 0]  CenterOfMassUnits=m  MomentsOfInertia=[1 1 1]  MomentsOfInertiaUnits=kg*m^2  ProductsOfInertia=[0 0 0]  ProductsOfInertiaUnits=kg*m^2  GraphicType=Marker  MarkerShape=Inertia  MarkerSize=20  GraphicVisPropType=SimpleVisualProperties  GraphicDiffuseColor=[0.5 0.5 0.5]  GraphicOpacity=0  GraphicSpecularColor=[0.5 0.5 0.5 1.0]  GraphicAmbientColor=[0.15 0.15 0.15 1.0]  GraphicEmissiveColor=[0.0 0.0 0.0 1.0]  GraphicShininess=75
  LA to Bearing : Subsystem
  Revolute : Subsystem  mask(Revolute Joint with 1D connections){whl_init_spd_jnt=whl_init_spd_upr}
      mask prompts: whl_init_spd_jnt "Initial Wheel Speed (rad/s)"
      mask help: Multibody Revolute Joint with connection to 1D mechanical network. Specify initial speed of Revolute Joint.
      mask Display: image('sm_car_variant_revolute.png')
  Steering Arm : Suspension_Utilities/Cylinder Between Two Points  hp_b=(hp_la_out+0.5*(hp_spr_bot-hp_la_out)).*rhs_hp  hp_f=hp_upr_rod.*rhs_hp  Mass=0  clr_solid=clr_upr  opc_solid=opc_upr  rad_solid=radius_upr
  Transform Align for Universal Joint : Suspension_Utilities/Transform Align Axis Two Points  hp_b=(hp_la_out+0.5*(hp_spr_bot-hp_la_out)).*rhs_hp  hp_t=hp_upr_rod.*rhs_hp  popup_f_axis=+Z
  Transform AxleCtr : sm_lib/Frames and Transforms/Rigid Transform  RotationMethod=None  FollAlignAxisA=+X  BaseAlignAxisA=+Y  FollAlignAxisB=+Y  BaseAlignAxisB=+Z  RotationStandardAxis=+Z  RotationAngle=0  RotationAngleUnits=deg  RotationArbitraryAxis=[0 0 1]  RotationSequenceAxes=FollowerAxes  RotationSequence=XYX  RotationSequenceAngles=[0 0 0]  RotationSequenceAnglesUnits=deg  RotationMatrix=[1 0 0; 0 1 0; 0 0 1]  Quaternion=[1 0 0 0]  TranslationMethod=StandardAxis  TranslationCartesianOffset=[0 0 0]  TranslationCartesianOffsetUnits=m  TranslationStandardAxis=-Z  TranslationStandardOffset=axle_len*rhs_upr/2  TranslationStandardOffsetUnits=m  TranslationROffset=0  TranslationROffsetUnits=m  TranslationThetaOffset=0  TranslationThetaOffsetUnits=deg  TranslationZOffset=0  TranslationZOffsetUnits=m
  Transform AxleIn : sm_lib/Frames and Transforms/Rigid Transform  RotationMethod=None  FollAlignAxisA=+X  BaseAlignAxisA=+Y  FollAlignAxisB=+Y  BaseAlignAxisB=+Z  RotationStandardAxis=+Z  RotationAngle=0  RotationAngleUnits=deg  RotationArbitraryAxis=[0 0 1]  RotationSequenceAxes=FollowerAxes  RotationSequence=XYX  RotationSequenceAngles=[0 0 0]  RotationSequenceAnglesUnits=deg  RotationMatrix=[1 0 0; 0 1 0; 0 0 1]  Quaternion=[1 0 0 0]  TranslationMethod=StandardAxis  TranslationCartesianOffset=[0 0 0]  TranslationCartesianOffsetUnits=m  TranslationStandardAxis=-Z  TranslationStandardOffset=axle_len*rhs_upr/2  TranslationStandardOffsetUnits=m  TranslationROffset=0  TranslationROffsetUnits=m  TranslationThetaOffset=0  TranslationThetaOffsetUnits=deg  TranslationZOffset=0  TranslationZOffsetUnits=m
  Transform Bearing to WC : sm_lib/Frames and Transforms/Rigid Transform  RotationMethod=None  FollAlignAxisA=+X  BaseAlignAxisA=+Y  FollAlignAxisB=+Y  BaseAlignAxisB=+Z  RotationStandardAxis=+Z  RotationAngle=0  RotationAngleUnits=deg  RotationArbitraryAxis=[0 0 1]  RotationSequenceAxes=FollowerAxes  RotationSequence=XYX  RotationSequenceAngles=[0 0 0]  RotationSequenceAnglesUnits=deg  RotationMatrix=[1 0 0; 0 1 0; 0 0 1]  Quaternion=[1 0 0 0]  TranslationMethod=StandardAxis  TranslationCartesianOffset=[0 0 0]  TranslationCartesianOffsetUnits=m  TranslationStandardAxis=+Z  TranslationStandardOffset=axle_whlc_to_bearing*rhs_upr  TranslationStandardOffsetUnits=m  TranslationROffset=0  TranslationROffsetUnits=m  TranslationThetaOffset=0  TranslationThetaOffsetUnits=deg  TranslationZOffset=0  TranslationZOffsetUnits=m
  Transform Upright CG : sm_lib/Frames and Transforms/Rigid Transform  RotationMethod=None  FollAlignAxisA=+X  BaseAlignAxisA=+Y  FollAlignAxisB=+Y  BaseAlignAxisB=+Z  RotationStandardAxis=+Z  RotationAngle=0.0  RotationAngleUnits=deg  RotationArbitraryAxis=[0 0 1]  RotationSequenceAxes=FollowerAxes  RotationSequence=XYX  RotationSequenceAngles=[0 0 0]  RotationSequenceAnglesUnits=deg  RotationMatrix=[1 0 0; 0 1 0; 0 0 1]  Quaternion=[1 0 0 0]  TranslationMethod=Cartesian  TranslationCartesianOffset=(hp_upr_cg-hp_la_out) .* [1, rhs_upr, 1]  TranslationCartesianOffsetUnits=m  TranslationStandardAxis=+Z  TranslationStandardOffset=0  TranslationStandardOffsetUnits=m  TranslationROffset=0  TranslationROffsetUnits=m  TranslationThetaOffset=0  TranslationThetaOffsetUnits=deg  TranslationZOffset=0  TranslationZOffsetUnits=m
  Transform Upright Ctr : sm_lib/Frames and Transforms/Rigid Transform  RotationMethod=None  FollAlignAxisA=+X  BaseAlignAxisA=+Y  FollAlignAxisB=+Y  BaseAlignAxisB=+Z  RotationStandardAxis=+Z  RotationAngle=0.0  RotationAngleUnits=deg  RotationArbitraryAxis=[0 0 1]  RotationSequenceAxes=FollowerAxes  RotationSequence=XYX  RotationSequenceAngles=[0 0 0]  RotationSequenceAnglesUnits=deg  RotationMatrix=[1 0 0; 0 1 0; 0 0 1]  Quaternion=[1 0 0 0]  TranslationMethod=Cartesian  TranslationCartesianOffset=0.5*(hp_spr_bot-hp_la_out).*rhs_hp  TranslationCartesianOffsetUnits=m  TranslationStandardAxis=+Z  TranslationStandardOffset=0  TranslationStandardOffsetUnits=m  TranslationROffset=0  TranslationROffsetUnits=m  TranslationThetaOffset=0  TranslationThetaOffsetUnits=deg  TranslationZOffset=0  TranslationZOffsetUnits=m
  Upright : Suspension_Utilities/Cylinder Between Two Points  hp_b=hp_la_out.*rhs_hp  hp_f=hp_spr_bot.*rhs_hp  Mass=0  clr_solid=clr_upr  opc_solid=opc_upr  rad_solid=radius_upr
  Vis Upright ARB : sm_lib/Body Elements/Spherical Solid  SphereRadius=size_conn_upr  SphereRadiusUnits=m  ExportEntireGeometry=off  InertiaType=PointMass  BasedOnType=Density  Density=0  DensityUnits=kg/m^3  Mass=0  MassUnits=kg  CenterOfMass=[0 0 0]  CenterOfMassUnits=m  MomentsOfInertia=[1 1 1]  MomentsOfInertiaUnits=kg*m^2  ProductsOfInertia=[0 0 0]  ProductsOfInertiaUnits=kg*m^2  GraphicType=FromGeometry  MarkerShape=Sphere  MarkerSize=10  GraphicVisPropType=SimpleVisualProperties  GraphicDiffuseColor=clr_conn_upr  GraphicOpacity=opc_conn_upr  GraphicSpecularColor=[0.5 0.5 0.5 1.0]  GraphicAmbientColor=[0.15 0.15 0.15 1.0]  GraphicEmissiveColor=[0.0 0.0 0.0 1.0]  GraphicShininess=75  DoExposeReferenceFrame=on  SerializedFrames=<Frames/>
  Vis Upright LA : sm_lib/Body Elements/Spherical Solid  SphereRadius=size_conn_upr  SphereRadiusUnits=m  ExportEntireGeometry=off  InertiaType=PointMass  BasedOnType=Density  Density=0  DensityUnits=kg/m^3  Mass=0  MassUnits=kg  CenterOfMass=[0 0 0]  CenterOfMassUnits=m  MomentsOfInertia=[1 1 1]  MomentsOfInertiaUnits=kg*m^2  ProductsOfInertia=[0 0 0]  ProductsOfInertiaUnits=kg*m^2  GraphicType=FromGeometry  MarkerShape=Sphere  MarkerSize=10  GraphicVisPropType=SimpleVisualProperties  GraphicDiffuseColor=clr_conn_upr  GraphicOpacity=opc_conn_upr  GraphicSpecularColor=[0.5 0.5 0.5 1.0]  GraphicAmbientColor=[0.15 0.15 0.15 1.0]  GraphicEmissiveColor=[0.0 0.0 0.0 1.0]  GraphicShininess=75  DoExposeReferenceFrame=on  SerializedFrames=<Frames/>
  Vis Upright UA : sm_lib/Body Elements/Spherical Solid  SphereRadius=size_conn_upr  SphereRadiusUnits=m  ExportEntireGeometry=off  InertiaType=PointMass  BasedOnType=Density  Density=0  DensityUnits=kg/m^3  Mass=0  MassUnits=kg  CenterOfMass=[0 0 0]  CenterOfMassUnits=m  MomentsOfInertia=[1 1 1]  MomentsOfInertiaUnits=kg*m^2  ProductsOfInertia=[0 0 0]  ProductsOfInertiaUnits=kg*m^2  GraphicType=FromGeometry  MarkerShape=Sphere  MarkerSize=10  GraphicVisPropType=SimpleVisualProperties  GraphicDiffuseColor=clr_conn_upr  GraphicOpacity=opc_conn_upr  GraphicSpecularColor=[0.5 0.5 0.5 1.0]  GraphicAmbientColor=[0.15 0.15 0.15 1.0]  GraphicEmissiveColor=[0.0 0.0 0.0 1.0]  GraphicShininess=75  DoExposeReferenceFrame=on  SerializedFrames=<Frames/>
  Vis Wheel Center : sm_lib/Body Elements/Spherical Solid  SphereRadius=size_conn_upr  SphereRadiusUnits=m  ExportEntireGeometry=off  InertiaType=PointMass  BasedOnType=Density  Density=0  DensityUnits=kg/m^3  Mass=0  MassUnits=kg  CenterOfMass=[0 0 0]  CenterOfMassUnits=m  MomentsOfInertia=[1 1 1]  MomentsOfInertiaUnits=kg*m^2  ProductsOfInertia=[0 0 0]  ProductsOfInertiaUnits=kg*m^2  GraphicType=FromGeometry  MarkerShape=Sphere  MarkerSize=10  GraphicVisPropType=SimpleVisualProperties  GraphicDiffuseColor=clr_conn_upr  GraphicOpacity=opc_conn_upr  GraphicSpecularColor=[0.5 0.5 0.5 1.0]  GraphicAmbientColor=[0.15 0.15 0.15 1.0]  GraphicEmissiveColor=[0.0 0.0 0.0 1.0]  GraphicShininess=75  DoExposeReferenceFrame=on  SerializedFrames=<Frames/>
  WhlCtr : PMIOPort  Side=Left
  RaceSpin : PMIOPort  Port=2  Side=Left
  RaceFix : PMIOPort  Port=3  Side=Left
  Axle1D : PMIOPort  Port=4  Side=Left
  AxleIn : PMIOPort  Port=5  Side=Left
  Rod : PMIOPort  Port=6  Side=Right
  sBot : PMIOPort  Port=7  Side=Right
  LA : PMIOPort  Port=8  Side=Right
  AR : PMIOPort  Port=9  Side=Right
  Out Bus Element : Outport  VectorParamsAs1DForOutWhenUnconnected=off  PortName=m  Element=Upright
  wires:
  Revolute/1(m) -> Out Bus Element/1
  connections:
  ARB/RConn1 -- AR/RConn1 -- Vis Upright ARB/RConn1
  AxleIn/RConn1 -- Transform AxleIn/RConn1
  Transform AxleCtr/RConn1 -- Transform AxleIn/LConn1 -- Axle/RConn1
  Transform Bearing to WC/LConn1 -- Revolute/LConn2 -- RaceSpin/RConn1
  Bearing Carrier/RConn1 -- Revolute/RConn1 -- RaceFix/RConn1 -- LA to Bearing/LConn1
  Transform Align for Universal Joint/LConn1 -- Steering Arm/RConn1
  Rod/RConn1 -- Transform Align for Universal Joint/RConn1
  Steering Arm/LConn1 -- Transform Upright Ctr/RConn1
  Transform Upright CG/RConn1 -- Inertia CG/RConn1
  sBot/RConn1 -- ARB/LConn1 -- Upright/RConn1 -- Vis Upright UA/RConn1
  Vis Upright LA/RConn1 -- Transform Upright CG/LConn1 -- LA to Bearing/RConn1 -- Upright/LConn1 -- Transform Upright Ctr/LConn1 -- LA/RConn1
  Transform Bearing to WC/RConn1 -- Transform AxleCtr/LConn1 -- WhlCtr/RConn1 -- Vis Wheel Center/RConn1
  Revolute/LConn1 -- Axle1D/RConn1
